simulink model "r2_b16a4x64f"  (R2012b)
settings: Solver=VariableStepDiscrete  SolverMode=SingleTasking  StartTime=0.0  StopTime=1  RelTol=1e-3
undefined symbols (not defined in the file): fft_stages, n_bits_ants, n_bits_xengs
libraries: xbsIndex_r4 x26846, casper_library_misc x230, xbsReplacements_r4 x24, casper_library_delays x8, xps_library x5, casper_library_communications x4
(part 25 of 227)

== system r2_b16a4x64f/vacc_monitor3 ==
  cnt_rst : Inport
  eof : Inport  Port=2
  error : Inport  Port=3
  Delay1 : Subsystem  AncestorBlock=casper_library_delays/pipeline  mask(pipeline){latency=2}
      mask help:
      | An explicitly laid-out delay line to avoid mapping to SRL16s
      | for use in pipelining to help achieve timing closure.
      mask init:
      | pipeline_init(gcb,'latency',latency);
      settings: AttributesFormatString=Latency = %<latency>
      mask Display:
      | port_label('input', 1, 'd');
      | port_label('output', 1, 'q');
      | disp(['Z^-', num2str(latency)]);
  Delay2 : Subsystem  AncestorBlock=casper_library_delays/pipeline  mask(pipeline){latency=2}
      mask help:
      | An explicitly laid-out delay line to avoid mapping to SRL16s
      | for use in pipelining to help achieve timing closure.
      mask init:
      | pipeline_init(gcb,'latency',latency);
      settings: AttributesFormatString=Latency = %<latency>
      mask Display:
      | port_label('input', 1, 'd');
      | port_label('output', 1, 'q');
      | disp(['Z^-', num2str(latency)]);
  Delay29 : Subsystem  AncestorBlock=casper_library_delays/pipeline  mask(pipeline){latency=2}
      mask help:
      | An explicitly laid-out delay line to avoid mapping to SRL16s
      | for use in pipelining to help achieve timing closure.
      mask init:
      | pipeline_init(gcb,'latency',latency);
      settings: AttributesFormatString=Latency = %<latency>
      mask Display:
      | port_label('input', 1, 'd');
      | port_label('output', 1, 'q');
      | disp(['Z^-', num2str(latency)]);
  Delay3 : Subsystem  AncestorBlock=casper_library_delays/pipeline  mask(pipeline){latency=2}
      mask help:
      | An explicitly laid-out delay line to avoid mapping to SRL16s
      | for use in pipelining to help achieve timing closure.
      mask init:
      | pipeline_init(gcb,'latency',latency);
      settings: AttributesFormatString=Latency = %<latency>
      mask Display:
      | port_label('input', 1, 'd');
      | port_label('output', 1, 'q');
      | disp(['Z^-', num2str(latency)]);
  Delay4 : Subsystem  AncestorBlock=casper_library_delays/pipeline  mask(pipeline){latency=2}
      mask help:
      | An explicitly laid-out delay line to avoid mapping to SRL16s
      | for use in pipelining to help achieve timing closure.
      mask init:
      | pipeline_init(gcb,'latency',latency);
      settings: AttributesFormatString=Latency = %<latency>
      mask Display:
      | port_label('input', 1, 'd');
      | port_label('output', 1, 'q');
      | disp(['Z^-', num2str(latency)]);
  payload_cnt1 : xbsIndex_r4/Counter  cnt_type=Free Running  cnt_to=0  operation=Up  start_count=0  cnt_by_val=1  arith_type=Unsigned  n_bits=16  bin_pt=0  load_pin=off  rst=on  en=on  explicit_period=off  period=1  dbl_ovrd=off  use_behavioral_HDL=on  implementation=Fabric  use_rpm=on  block_type=counter
      settings: xl_area=[0, 0, 0, 0, 0, 0, 0]
  payload_cnt3 : xbsIndex_r4/Counter  cnt_type=Free Running  cnt_to=0  operation=Up  start_count=0  cnt_by_val=1  arith_type=Unsigned  n_bits=16  bin_pt=0  load_pin=off  rst=on  en=on  explicit_period=off  period=1  dbl_ovrd=off  use_behavioral_HDL=on  implementation=Fabric  use_rpm=on  block_type=counter
      settings: xl_area=[0, 0, 0, 0, 0, 0, 0]
  pkt_cnt : Outport
  error_cnt : Outport  Port=2
  wires:
  Delay3/1(q) -> pkt_cnt/1
  error/1 -> Delay29/1(d)
  Delay4/1(q) -> error_cnt/1
  eof/1 -> Delay1/1(d)
  cnt_rst/1 -> Delay2/1(d)
  payload_cnt1/1 -> Delay4/1(d)
  Delay29/1(q) -> payload_cnt1/2
  Delay1/1(q) -> payload_cnt3/2
  Delay2/1(q) -> payload_cnt1/1, payload_cnt3/1
  payload_cnt3/1 -> Delay3/1(d)

== system r2_b16a4x64f/vacc_monitor4 ==
  cnt_rst : Inport
  new_acc : Inport  Port=2
  ready : Inport  Port=3
  eof : Inport  Port=4
  error : Inport  Port=5
  Delay1 : Subsystem  AncestorBlock=casper_library_delays/pipeline  mask(pipeline){latency=2}
      mask help:
      | An explicitly laid-out delay line to avoid mapping to SRL16s
      | for use in pipelining to help achieve timing closure.
      mask init:
      | pipeline_init(gcb,'latency',latency);
      settings: AttributesFormatString=Latency = %<latency>
      mask Display:
      | port_label('input', 1, 'd');
      | port_label('output', 1, 'q');
      | disp(['Z^-', num2str(latency)]);
  Delay121 : Subsystem  AncestorBlock=casper_library_delays/pipeline  mask(pipeline){latency=2}
      mask help:
      | An explicitly laid-out delay line to avoid mapping to SRL16s
      | for use in pipelining to help achieve timing closure.
      mask init:
      | pipeline_init(gcb,'latency',latency);
      settings: AttributesFormatString=Latency = %<latency>
      mask Display:
      | port_label('input', 1, 'd');
      | port_label('output', 1, 'q');
      | disp(['Z^-', num2str(latency)]);
  Delay2 : Subsystem  AncestorBlock=casper_library_delays/pipeline  mask(pipeline){latency=2}
      mask help:
      | An explicitly laid-out delay line to avoid mapping to SRL16s
      | for use in pipelining to help achieve timing closure.
      mask init:
      | pipeline_init(gcb,'latency',latency);
      settings: AttributesFormatString=Latency = %<latency>
      mask Display:
      | port_label('input', 1, 'd');
      | port_label('output', 1, 'q');
      | disp(['Z^-', num2str(latency)]);
  Delay25 : Subsystem  AncestorBlock=casper_library_delays/pipeline  mask(pipeline){latency=2}
      mask help:
      | An explicitly laid-out delay line to avoid mapping to SRL16s
      | for use in pipelining to help achieve timing closure.
      mask init:
      | pipeline_init(gcb,'latency',latency);
      settings: AttributesFormatString=Latency = %<latency>
      mask Display:
      | port_label('input', 1, 'd');
      | port_label('output', 1, 'q');
      | disp(['Z^-', num2str(latency)]);
  Delay3 : Subsystem  AncestorBlock=casper_library_delays/pipeline  mask(pipeline){latency=2}
      mask help:
      | An explicitly laid-out delay line to avoid mapping to SRL16s
      | for use in pipelining to help achieve timing closure.
      mask init:
      | pipeline_init(gcb,'latency',latency);
      settings: AttributesFormatString=Latency = %<latency>
      mask Display:
      | port_label('input', 1, 'd');
      | port_label('output', 1, 'q');
      | disp(['Z^-', num2str(latency)]);
  Delay4 : Subsystem  AncestorBlock=casper_library_delays/pipeline  mask(pipeline){latency=2}
      mask help:
      | An explicitly laid-out delay line to avoid mapping to SRL16s
      | for use in pipelining to help achieve timing closure.
      mask init:
      | pipeline_init(gcb,'latency',latency);
      settings: AttributesFormatString=Latency = %<latency>
      mask Display:
      | port_label('input', 1, 'd');
      | port_label('output', 1, 'q');
      | disp(['Z^-', num2str(latency)]);
  Delay5 : Subsystem  AncestorBlock=casper_library_delays/pipeline  mask(pipeline){latency=2}
      mask help:
      | An explicitly laid-out delay line to avoid mapping to SRL16s
      | for use in pipelining to help achieve timing closure.
      mask init:
      | pipeline_init(gcb,'latency',latency);
      settings: AttributesFormatString=Latency = %<latency>
      mask Display:
      | port_label('input', 1, 'd');
      | port_label('output', 1, 'q');
      | disp(['Z^-', num2str(latency)]);
  Delay6 : Subsystem  AncestorBlock=casper_library_delays/pipeline  mask(pipeline){latency=2}
      mask help:
      | An explicitly laid-out delay line to avoid mapping to SRL16s
      | for use in pipelining to help achieve timing closure.
      mask init:
      | pipeline_init(gcb,'latency',latency);
      settings: AttributesFormatString=Latency = %<latency>
      mask Display:
      | port_label('input', 1, 'd');
      | port_label('output', 1, 'q');
      | disp(['Z^-', num2str(latency)]);
  Delay7 : Subsystem  AncestorBlock=casper_library_delays/pipeline  mask(pipeline){latency=2}
      mask help:
      | An explicitly laid-out delay line to avoid mapping to SRL16s
      | for use in pipelining to help achieve timing closure.
      mask init:
      | pipeline_init(gcb,'latency',latency);
      settings: AttributesFormatString=Latency = %<latency>
      mask Display:
      | port_label('input', 1, 'd');
      | port_label('output', 1, 'q');
      | disp(['Z^-', num2str(latency)]);
  payload_cnt{1..4} (4 alike) : xbsIndex_r4/Counter  cnt_type=Free Running  cnt_to=0  operation=Up  start_count=0  cnt_by_val=1  arith_type=Unsigned  n_bits=16  bin_pt=0  load_pin=off  rst=on  en=on  explicit_period=off  period=1  dbl_ovrd=off  use_behavioral_HDL=on  implementation=Fabric  use_rpm=on  block_type=counter
      settings: xl_area=[0, 0, 0, 0, 0, 0, 0]
  acc_cnt : Outport
  ready_cnt : Outport  Port=2
  eof_cnt : Outport  Port=3
  error_cnt : Outport  Port=4
  wires:
  Delay5/1(q) -> eof_cnt/1
  Delay4/1(q) -> ready_cnt/1
  Delay7/1(q) -> payload_cnt2/2
  Delay6/1(q) -> payload_cnt4/2
  payload_cnt4/1 -> Delay5/1(d)
  payload_cnt2/1 -> Delay4/1(d)
  ready/1 -> Delay7/1(d)
  eof/1 -> Delay6/1(d)
  Delay3/1(q) -> payload_cnt3/1, payload_cnt2/1, payload_cnt4/1, payload_cnt1/1
  Delay121/1(q) -> acc_cnt/1
  error/1 -> Delay1/1(d)
  Delay25/1(q) -> error_cnt/1
  new_acc/1 -> Delay2/1(d)
  cnt_rst/1 -> Delay3/1(d)
  payload_cnt1/1 -> Delay25/1(d)
  Delay1/1(q) -> payload_cnt1/2
  payload_cnt3/1 -> Delay121/1(d)
  Delay2/1(q) -> payload_cnt3/2

== system r2_b16a4x64f/vacc_monitor5 ==
  cnt_rst : Inport
  eof : Inport  Port=2
  error : Inport  Port=3
  Delay1 : Subsystem  AncestorBlock=casper_library_delays/pipeline  mask(pipeline){latency=2}
      mask help:
      | An explicitly laid-out delay line to avoid mapping to SRL16s
      | for use in pipelining to help achieve timing closure.
      mask init:
      | pipeline_init(gcb,'latency',latency);
      settings: AttributesFormatString=Latency = %<latency>
      mask Display:
      | port_label('input', 1, 'd');
      | port_label('output', 1, 'q');
      | disp(['Z^-', num2str(latency)]);
  Delay2 : Subsystem  AncestorBlock=casper_library_delays/pipeline  mask(pipeline){latency=2}
      mask help:
      | An explicitly laid-out delay line to avoid mapping to SRL16s
      | for use in pipelining to help achieve timing closure.
      mask init:
      | pipeline_init(gcb,'latency',latency);
      settings: AttributesFormatString=Latency = %<latency>
      mask Display:
      | port_label('input', 1, 'd');
      | port_label('output', 1, 'q');
      | disp(['Z^-', num2str(latency)]);
  Delay29 : Subsystem  AncestorBlock=casper_library_delays/pipeline  mask(pipeline){latency=2}
      mask help:
      | An explicitly laid-out delay line to avoid mapping to SRL16s
      | for use in pipelining to help achieve timing closure.
      mask init:
      | pipeline_init(gcb,'latency',latency);
      settings: AttributesFormatString=Latency = %<latency>
      mask Display:
      | port_label('input', 1, 'd');
      | port_label('output', 1, 'q');
      | disp(['Z^-', num2str(latency)]);
  Delay3 : Subsystem  AncestorBlock=casper_library_delays/pipeline  mask(pipeline){latency=2}
      mask help:
      | An explicitly laid-out delay line to avoid mapping to SRL16s
      | for use in pipelining to help achieve timing closure.
      mask init:
      | pipeline_init(gcb,'latency',latency);
      settings: AttributesFormatString=Latency = %<latency>
      mask Display:
      | port_label('input', 1, 'd');
      | port_label('output', 1, 'q');
      | disp(['Z^-', num2str(latency)]);
  Delay4 : Subsystem  AncestorBlock=casper_library_delays/pipeline  mask(pipeline){latency=2}
      mask help:
      | An explicitly laid-out delay line to avoid mapping to SRL16s
      | for use in pipelining to help achieve timing closure.
      mask init:
      | pipeline_init(gcb,'latency',latency);
      settings: AttributesFormatString=Latency = %<latency>
      mask Display:
      | port_label('input', 1, 'd');
      | port_label('output', 1, 'q');
      | disp(['Z^-', num2str(latency)]);
  payload_cnt1 : xbsIndex_r4/Counter  cnt_type=Free Running  cnt_to=0  operation=Up  start_count=0  cnt_by_val=1  arith_type=Unsigned  n_bits=16  bin_pt=0  load_pin=off  rst=on  en=on  explicit_period=off  period=1  dbl_ovrd=off  use_behavioral_HDL=on  implementation=Fabric  use_rpm=on  block_type=counter
      settings: xl_area=[0, 0, 0, 0, 0, 0, 0]
  payload_cnt3 : xbsIndex_r4/Counter  cnt_type=Free Running  cnt_to=0  operation=Up  start_count=0  cnt_by_val=1  arith_type=Unsigned  n_bits=16  bin_pt=0  load_pin=off  rst=on  en=on  explicit_period=off  period=1  dbl_ovrd=off  use_behavioral_HDL=on  implementation=Fabric  use_rpm=on  block_type=counter
      settings: xl_area=[0, 0, 0, 0, 0, 0, 0]
  pkt_cnt : Outport
  error_cnt : Outport  Port=2
  wires:
  Delay3/1(q) -> pkt_cnt/1
  error/1 -> Delay29/1(d)
  Delay4/1(q) -> error_cnt/1
  eof/1 -> Delay1/1(d)
  cnt_rst/1 -> Delay2/1(d)
  payload_cnt1/1 -> Delay4/1(d)
  Delay29/1(q) -> payload_cnt1/2
  Delay1/1(q) -> payload_cnt3/2
  Delay2/1(q) -> payload_cnt1/1, payload_cnt3/1
  payload_cnt3/1 -> Delay3/1(d)

== system r2_b16a4x64f/vacc_monitor6 ==
  cnt_rst : Inport
  cal : Inport  Port=2
  inof : Inport  Port=3
  rst : Inport  Port=4
  outof : Inport  Port=5
  parity : Inport  Port=6
  Delay1 : Subsystem  AncestorBlock=casper_library_delays/pipeline  mask(pipeline){latency=2}
      mask help:
      | An explicitly laid-out delay line to avoid mapping to SRL16s
      | for use in pipelining to help achieve timing closure.
      mask init:
      | pipeline_init(gcb,'latency',latency);
      settings: AttributesFormatString=Latency = %<latency>
      mask Display:
      | port_label('input', 1, 'd');
      | port_label('output', 1, 'q');
      | disp(['Z^-', num2str(latency)]);
  Delay2 : Subsystem  AncestorBlock=casper_library_delays/pipeline  mask(pipeline){latency=2}
      mask help:
      | An explicitly laid-out delay line to avoid mapping to SRL16s
      | for use in pipelining to help achieve timing closure.
      mask init:
      | pipeline_init(gcb,'latency',latency);
      settings: AttributesFormatString=Latency = %<latency>
      mask Display:
      | port_label('input', 1, 'd');
      | port_label('output', 1, 'q');
      | disp(['Z^-', num2str(latency)]);
  Delay25 : Subsystem  AncestorBlock=casper_library_delays/pipeline  mask(pipeline){latency=2}
      mask help:
      | An explicitly laid-out delay line to avoid mapping to SRL16s
      | for use in pipelining to help achieve timing closure.
      mask init:
      | pipeline_init(gcb,'latency',latency);
      settings: AttributesFormatString=Latency = %<latency>
      mask Display:
      | port_label('input', 1, 'd');
      | port_label('output', 1, 'q');
      | disp(['Z^-', num2str(latency)]);
  Delay3 : Subsystem  AncestorBlock=casper_library_delays/pipeline  mask(pipeline){latency=2}
      mask help:
      | An explicitly laid-out delay line to avoid mapping to SRL16s
      | for use in pipelining to help achieve timing closure.
      mask init:
      | pipeline_init(gcb,'latency',latency);
      settings: AttributesFormatString=Latency = %<latency>
      mask Display:
      | port_label('input', 1, 'd');
      | port_label('output', 1, 'q');
      | disp(['Z^-', num2str(latency)]);
  Delay4 : Subsystem  AncestorBlock=casper_library_delays/pipeline  mask(pipeline){latency=2}
      mask help:
      | An explicitly laid-out delay line to avoid mapping to SRL16s
      | for use in pipelining to help achieve timing closure.
      mask init:
      | pipeline_init(gcb,'latency',latency);
      settings: AttributesFormatString=Latency = %<latency>
      mask Display:
      | port_label('input', 1, 'd');
      | port_label('output', 1, 'q');
      | disp(['Z^-', num2str(latency)]);
  payload_cnt{1..5} (5 alike) : xbsIndex_r4/Counter  cnt_type=Free Running  cnt_to=0  operation=Up  start_count=0  cnt_by_val=1  arith_type=Unsigned  n_bits=6  bin_pt=0  load_pin=off  rst=on  en=on  explicit_period=off  period=1  dbl_ovrd=off  use_behavioral_HDL=off  implementation=Fabric  use_rpm=on  block_type=counter
      settings: xl_area=[0, 0, 0, 0, 0, 0, 0]
  cal_cnt : Outport
  inof_cnt : Outport  Port=2
  rst_cnt : Outport  Port=3
  outof_cnt : Outport  Port=4
  parity_cnt : Outport  Port=5
  wires:
  Delay25/1(q) -> cal_cnt/1
  inof/1 -> payload_cnt3/2
  cnt_rst/1 -> payload_cnt1/1, payload_cnt2/1, payload_cnt4/1, payload_cnt5/1, payload_cnt3/1
  payload_cnt1/1 -> Delay25/1(d)
  cal/1 -> payload_cnt1/2
  payload_cnt3/1 -> Delay1/1(d)
  rst/1 -> payload_cnt2/2
  outof/1 -> payload_cnt4/2
  payload_cnt2/1 -> Delay2/1(d)
  payload_cnt4/1 -> Delay3/1(d)
  parity/1 -> payload_cnt5/2
  payload_cnt5/1 -> Delay4/1(d)
  Delay1/1(q) -> inof_cnt/1
  Delay2/1(q) -> rst_cnt/1
  Delay3/1(q) -> outof_cnt/1
  Delay4/1(q) -> parity_cnt/1

== system r2_b16a4x64f/vacc_monitor7 ==
  cnt_rst : Inport
  eof : Inport  Port=2
  error : Inport  Port=3
  Delay1 : Subsystem  AncestorBlock=casper_library_delays/pipeline  mask(pipeline){latency=2}
      mask help:
      | An explicitly laid-out delay line to avoid mapping to SRL16s
      | for use in pipelining to help achieve timing closure.
      mask init:
      | pipeline_init(gcb,'latency',latency);
      settings: AttributesFormatString=Latency = %<latency>
      mask Display:
      | port_label('input', 1, 'd');
      | port_label('output', 1, 'q');
      | disp(['Z^-', num2str(latency)]);
  Delay2 : Subsystem  AncestorBlock=casper_library_delays/pipeline  mask(pipeline){latency=2}
      mask help:
      | An explicitly laid-out delay line to avoid mapping to SRL16s
      | for use in pipelining to help achieve timing closure.
      mask init:
      | pipeline_init(gcb,'latency',latency);
      settings: AttributesFormatString=Latency = %<latency>
      mask Display:
      | port_label('input', 1, 'd');
      | port_label('output', 1, 'q');
      | disp(['Z^-', num2str(latency)]);
  Delay29 : Subsystem  AncestorBlock=casper_library_delays/pipeline  mask(pipeline){latency=2}
      mask help:
      | An explicitly laid-out delay line to avoid mapping to SRL16s
      | for use in pipelining to help achieve timing closure.
      mask init:
      | pipeline_init(gcb,'latency',latency);
      settings: AttributesFormatString=Latency = %<latency>
      mask Display:
      | port_label('input', 1, 'd');
      | port_label('output', 1, 'q');
      | disp(['Z^-', num2str(latency)]);
  Delay3 : Subsystem  AncestorBlock=casper_library_delays/pipeline  mask(pipeline){latency=2}
      mask help:
      | An explicitly laid-out delay line to avoid mapping to SRL16s
      | for use in pipelining to help achieve timing closure.
      mask init:
      | pipeline_init(gcb,'latency',latency);
      settings: AttributesFormatString=Latency = %<latency>
      mask Display:
      | port_label('input', 1, 'd');
      | port_label('output', 1, 'q');
      | disp(['Z^-', num2str(latency)]);
  Delay4 : Subsystem  AncestorBlock=casper_library_delays/pipeline  mask(pipeline){latency=2}
      mask help:
      | An explicitly laid-out delay line to avoid mapping to SRL16s
      | for use in pipelining to help achieve timing closure.
      mask init:
      | pipeline_init(gcb,'latency',latency);
      settings: AttributesFormatString=Latency = %<latency>
      mask Display:
      | port_label('input', 1, 'd');
      | port_label('output', 1, 'q');
      | disp(['Z^-', num2str(latency)]);
  payload_cnt1 : xbsIndex_r4/Counter  cnt_type=Free Running  cnt_to=0  operation=Up  start_count=0  cnt_by_val=1  arith_type=Unsigned  n_bits=16  bin_pt=0  load_pin=off  rst=on  en=on  explicit_period=off  period=1  dbl_ovrd=off  use_behavioral_HDL=on  implementation=Fabric  use_rpm=on  block_type=counter
      settings: xl_area=[0, 0, 0, 0, 0, 0, 0]
  payload_cnt3 : xbsIndex_r4/Counter  cnt_type=Free Running  cnt_to=0  operation=Up  start_count=0  cnt_by_val=1  arith_type=Unsigned  n_bits=16  bin_pt=0  load_pin=off  rst=on  en=on  explicit_period=off  period=1  dbl_ovrd=off  use_behavioral_HDL=on  implementation=Fabric  use_rpm=on  block_type=counter
      settings: xl_area=[0, 0, 0, 0, 0, 0, 0]
  pkt_cnt : Outport
  error_cnt : Outport  Port=2
  wires:
  payload_cnt3/1 -> Delay3/1(d)
  Delay2/1(q) -> payload_cnt3/1, payload_cnt1/1
  Delay1/1(q) -> payload_cnt3/2
  Delay29/1(q) -> payload_cnt1/2
  payload_cnt1/1 -> Delay4/1(d)
  cnt_rst/1 -> Delay2/1(d)
  eof/1 -> Delay1/1(d)
  Delay4/1(q) -> error_cnt/1
  error/1 -> Delay29/1(d)
  Delay3/1(q) -> pkt_cnt/1

== system r2_b16a4x64f/vacc_monitor8 ==
  cnt_rst : Inport
  cal : Inport  Port=2
  inof : Inport  Port=3
  rst : Inport  Port=4
  outof : Inport  Port=5
  parity : Inport  Port=6
  Delay1 : Subsystem  AncestorBlock=casper_library_delays/pipeline  mask(pipeline){latency=2}
      mask help:
      | An explicitly laid-out delay line to avoid mapping to SRL16s
      | for use in pipelining to help achieve timing closure.
      mask init:
      | pipeline_init(gcb,'latency',latency);
      settings: AttributesFormatString=Latency = %<latency>
      mask Display:
      | port_label('input', 1, 'd');
      | port_label('output', 1, 'q');
      | disp(['Z^-', num2str(latency)]);
  Delay10 : Subsystem  AncestorBlock=casper_library_delays/pipeline  mask(pipeline){latency=2}
      mask help:
      | An explicitly laid-out delay line to avoid mapping to SRL16s
      | for use in pipelining to help achieve timing closure.
      mask init:
      | pipeline_init(gcb,'latency',latency);
      settings: AttributesFormatString=Latency = %<latency>
      mask Display:
      | port_label('input', 1, 'd');
      | port_label('output', 1, 'q');
      | disp(['Z^-', num2str(latency)]);
  Delay2 : Subsystem  AncestorBlock=casper_library_delays/pipeline  mask(pipeline){latency=2}
      mask help:
      | An explicitly laid-out delay line to avoid mapping to SRL16s
      | for use in pipelining to help achieve timing closure.
      mask init:
      | pipeline_init(gcb,'latency',latency);
      settings: AttributesFormatString=Latency = %<latency>
      mask Display:
      | port_label('input', 1, 'd');
      | port_label('output', 1, 'q');
      | disp(['Z^-', num2str(latency)]);
  Delay29 : Subsystem  AncestorBlock=casper_library_delays/pipeline  mask(pipeline){latency=2}
      mask help:
      | An explicitly laid-out delay line to avoid mapping to SRL16s
      | for use in pipelining to help achieve timing closure.
      mask init:
      | pipeline_init(gcb,'latency',latency);
      settings: AttributesFormatString=Latency = %<latency>
      mask Display:
      | port_label('input', 1, 'd');
      | port_label('output', 1, 'q');
      | disp(['Z^-', num2str(latency)]);
  Delay3 : Subsystem  AncestorBlock=casper_library_delays/pipeline  mask(pipeline){latency=2}
      mask help:
      | An explicitly laid-out delay line to avoid mapping to SRL16s
      | for use in pipelining to help achieve timing closure.
      mask init:
      | pipeline_init(gcb,'latency',latency);
      settings: AttributesFormatString=Latency = %<latency>
      mask Display:
      | port_label('input', 1, 'd');
      | port_label('output', 1, 'q');
      | disp(['Z^-', num2str(latency)]);
  Delay4 : Subsystem  AncestorBlock=casper_library_delays/pipeline  mask(pipeline){latency=2}
      mask help:
      | An explicitly laid-out delay line to avoid mapping to SRL16s
      | for use in pipelining to help achieve timing closure.
      mask init:
      | pipeline_init(gcb,'latency',latency);
      settings: AttributesFormatString=Latency = %<latency>
      mask Display:
      | port_label('input', 1, 'd');
      | port_label('output', 1, 'q');
      | disp(['Z^-', num2str(latency)]);
  Delay5 : Subsystem  AncestorBlock=casper_library_delays/pipeline  mask(pipeline){latency=2}
      mask help:
      | An explicitly laid-out delay line to avoid mapping to SRL16s
      | for use in pipelining to help achieve timing closure.
      mask init:
      | pipeline_init(gcb,'latency',latency);
      settings: AttributesFormatString=Latency = %<latency>
      mask Display:
      | port_label('input', 1, 'd');
      | port_label('output', 1, 'q');
      | disp(['Z^-', num2str(latency)]);
  Delay6 : Subsystem  AncestorBlock=casper_library_delays/pipeline  mask(pipeline){latency=2}
      mask help:
      | An explicitly laid-out delay line to avoid mapping to SRL16s
      | for use in pipelining to help achieve timing closure.
      mask init:
      | pipeline_init(gcb,'latency',latency);
      settings: AttributesFormatString=Latency = %<latency>
      mask Display:
      | port_label('input', 1, 'd');
      | port_label('output', 1, 'q');
      | disp(['Z^-', num2str(latency)]);
  Delay7 : Subsystem  AncestorBlock=casper_library_delays/pipeline  mask(pipeline){latency=2}
      mask help:
      | An explicitly laid-out delay line to avoid mapping to SRL16s
      | for use in pipelining to help achieve timing closure.
      mask init:
      | pipeline_init(gcb,'latency',latency);
      settings: AttributesFormatString=Latency = %<latency>
      mask Display:
      | port_label('input', 1, 'd');
      | port_label('output', 1, 'q');
      | disp(['Z^-', num2str(latency)]);
  Delay8 : Subsystem  AncestorBlock=casper_library_delays/pipeline  mask(pipeline){latency=2}
      mask help:
      | An explicitly laid-out delay line to avoid mapping to SRL16s
      | for use in pipelining to help achieve timing closure.
      mask init:
      | pipeline_init(gcb,'latency',latency);
      settings: AttributesFormatString=Latency = %<latency>
      mask Display:
      | port_label('input', 1, 'd');
      | port_label('output', 1, 'q');
      | disp(['Z^-', num2str(latency)]);
  Delay9 : Subsystem  AncestorBlock=casper_library_delays/pipeline  mask(pipeline){latency=2}
      mask help:
      | An explicitly laid-out delay line to avoid mapping to SRL16s
      | for use in pipelining to help achieve timing closure.
      mask init:
      | pipeline_init(gcb,'latency',latency);
      settings: AttributesFormatString=Latency = %<latency>
      mask Display:
      | port_label('input', 1, 'd');
      | port_label('output', 1, 'q');
      | disp(['Z^-', num2str(latency)]);
  payload_cnt{1..5} (5 alike) : xbsIndex_r4/Counter  cnt_type=Free Running  cnt_to=0  operation=Up  start_count=0  cnt_by_val=1  arith_type=Unsigned  n_bits=6  bin_pt=0  load_pin=off  rst=on  en=on  explicit_period=off  period=1  dbl_ovrd=off  use_behavioral_HDL=off  implementation=Fabric  use_rpm=on  block_type=counter
      settings: xl_area=[0, 0, 0, 0, 0, 0, 0]
  cal_cnt : Outport
  inof_cnt : Outport  Port=2
  rst_cnt : Outport  Port=3
  outof_cnt : Outport  Port=4
  parity_cnt : Outport  Port=5
  wires:
  cal/1 -> Delay29/1(d)
  inof/1 -> Delay8/1(d)
  cnt_rst/1 -> Delay2/1(d)
  payload_cnt1/1 -> Delay1/1(d)
  Delay29/1(q) -> payload_cnt1/2
  rst/1 -> Delay7/1(d)
  outof/1 -> Delay9/1(d)
  parity/1 -> Delay10/1(d)
  Delay2/1(q) -> payload_cnt1/1, payload_cnt2/1, payload_cnt4/1, payload_cnt5/1, payload_cnt3/1
  payload_cnt3/1 -> Delay3/1(d)
  payload_cnt2/1 -> Delay4/1(d)
  payload_cnt4/1 -> Delay5/1(d)
  payload_cnt5/1 -> Delay6/1(d)
  Delay3/1(q) -> inof_cnt/1
  Delay1/1(q) -> cal_cnt/1
  Delay4/1(q) -> rst_cnt/1
  Delay5/1(q) -> outof_cnt/1
  Delay6/1(q) -> parity_cnt/1
  Delay10/1(q) -> payload_cnt5/2
  Delay9/1(q) -> payload_cnt4/2
  Delay7/1(q) -> payload_cnt2/2
  Delay8/1(q) -> payload_cnt3/2

== system r2_b16a4x64f/vacc_monitor9 ==
  cnt_rst : Inport
  cal : Inport  Port=2
  inof : Inport  Port=3
  rst : Inport  Port=4
  outof : Inport  Port=5
  parity : Inport  Port=6
  Delay1 : Subsystem  AncestorBlock=casper_library_delays/pipeline  mask(pipeline){latency=2}
      mask help:
      | An explicitly laid-out delay line to avoid mapping to SRL16s
      | for use in pipelining to help achieve timing closure.
      mask init:
      | pipeline_init(gcb,'latency',latency);
      settings: AttributesFormatString=Latency = %<latency>
      mask Display:
      | port_label('input', 1, 'd');
      | port_label('output', 1, 'q');
      | disp(['Z^-', num2str(latency)]);
  Delay10 : Subsystem  AncestorBlock=casper_library_delays/pipeline  mask(pipeline){latency=2}
      mask help:
      | An explicitly laid-out delay line to avoid mapping to SRL16s
      | for use in pipelining to help achieve timing closure.
      mask init:
      | pipeline_init(gcb,'latency',latency);
      settings: AttributesFormatString=Latency = %<latency>
      mask Display:
      | port_label('input', 1, 'd');
      | port_label('output', 1, 'q');
      | disp(['Z^-', num2str(latency)]);
  Delay2 : Subsystem  AncestorBlock=casper_library_delays/pipeline  mask(pipeline){latency=2}
      mask help:
      | An explicitly laid-out delay line to avoid mapping to SRL16s
      | for use in pipelining to help achieve timing closure.
      mask init:
      | pipeline_init(gcb,'latency',latency);
      settings: AttributesFormatString=Latency = %<latency>
      mask Display:
      | port_label('input', 1, 'd');
      | port_label('output', 1, 'q');
      | disp(['Z^-', num2str(latency)]);
  Delay29 : Subsystem  AncestorBlock=casper_library_delays/pipeline  mask(pipeline){latency=2}
      mask help:
      | An explicitly laid-out delay line to avoid mapping to SRL16s
      | for use in pipelining to help achieve timing closure.
      mask init:
      | pipeline_init(gcb,'latency',latency);
      settings: AttributesFormatString=Latency = %<latency>
      mask Display:
      | port_label('input', 1, 'd');
      | port_label('output', 1, 'q');
      | disp(['Z^-', num2str(latency)]);
  Delay3 : Subsystem  AncestorBlock=casper_library_delays/pipeline  mask(pipeline){latency=2}
      mask help:
      | An explicitly laid-out delay line to avoid mapping to SRL16s
      | for use in pipelining to help achieve timing closure.
      mask init:
      | pipeline_init(gcb,'latency',latency);
      settings: AttributesFormatString=Latency = %<latency>
      mask Display:
      | port_label('input', 1, 'd');
      | port_label('output', 1, 'q');
      | disp(['Z^-', num2str(latency)]);
  Delay4 : Subsystem  AncestorBlock=casper_library_delays/pipeline  mask(pipeline){latency=2}
      mask help:
      | An explicitly laid-out delay line to avoid mapping to SRL16s
      | for use in pipelining to help achieve timing closure.
      mask init:
      | pipeline_init(gcb,'latency',latency);
      settings: AttributesFormatString=Latency = %<latency>
      mask Display:
      | port_label('input', 1, 'd');
      | port_label('output', 1, 'q');
      | disp(['Z^-', num2str(latency)]);
  Delay5 : Subsystem  AncestorBlock=casper_library_delays/pipeline  mask(pipeline){latency=2}
      mask help:
      | An explicitly laid-out delay line to avoid mapping to SRL16s
      | for use in pipelining to help achieve timing closure.
      mask init:
      | pipeline_init(gcb,'latency',latency);
      settings: AttributesFormatString=Latency = %<latency>
      mask Display:
      | port_label('input', 1, 'd');
      | port_label('output', 1, 'q');
      | disp(['Z^-', num2str(latency)]);
  Delay6 : Subsystem  AncestorBlock=casper_library_delays/pipeline  mask(pipeline){latency=2}
      mask help:
      | An explicitly laid-out delay line to avoid mapping to SRL16s
      | for use in pipelining to help achieve timing closure.
      mask init:
      | pipeline_init(gcb,'latency',latency);
      settings: AttributesFormatString=Latency = %<latency>
      mask Display:
      | port_label('input', 1, 'd');
      | port_label('output', 1, 'q');
      | disp(['Z^-', num2str(latency)]);
  Delay7 : Subsystem  AncestorBlock=casper_library_delays/pipeline  mask(pipeline){latency=2}
      mask help:
      | An explicitly laid-out delay line to avoid mapping to SRL16s
      | for use in pipelining to help achieve timing closure.
      mask init:
      | pipeline_init(gcb,'latency',latency);
      settings: AttributesFormatString=Latency = %<latency>
      mask Display:
      | port_label('input', 1, 'd');
      | port_label('output', 1, 'q');
      | disp(['Z^-', num2str(latency)]);
  Delay8 : Subsystem  AncestorBlock=casper_library_delays/pipeline  mask(pipeline){latency=2}
      mask help:
      | An explicitly laid-out delay line to avoid mapping to SRL16s
      | for use in pipelining to help achieve timing closure.
      mask init:
      | pipeline_init(gcb,'latency',latency);
      settings: AttributesFormatString=Latency = %<latency>
      mask Display:
      | port_label('input', 1, 'd');
      | port_label('output', 1, 'q');
      | disp(['Z^-', num2str(latency)]);
  Delay9 : Subsystem  AncestorBlock=casper_library_delays/pipeline  mask(pipeline){latency=2}
      mask help:
      | An explicitly laid-out delay line to avoid mapping to SRL16s
      | for use in pipelining to help achieve timing closure.
      mask init:
      | pipeline_init(gcb,'latency',latency);
      settings: AttributesFormatString=Latency = %<latency>
      mask Display:
      | port_label('input', 1, 'd');
      | port_label('output', 1, 'q');
      | disp(['Z^-', num2str(latency)]);
  payload_cnt{1..5} (5 alike) : xbsIndex_r4/Counter  cnt_type=Free Running  cnt_to=0  operation=Up  start_count=0  cnt_by_val=1  arith_type=Unsigned  n_bits=6  bin_pt=0  load_pin=off  rst=on  en=on  explicit_period=off  period=1  dbl_ovrd=off  use_behavioral_HDL=off  implementation=Fabric  use_rpm=on  block_type=counter
      settings: xl_area=[0, 0, 0, 0, 0, 0, 0]
  cal_cnt : Outport
  inof_cnt : Outport  Port=2
  rst_cnt : Outport  Port=3
  outof_cnt : Outport  Port=4
  parity_cnt : Outport  Port=5
  wires:
  Delay8/1(q) -> payload_cnt3/2
  Delay7/1(q) -> payload_cnt2/2
  Delay9/1(q) -> payload_cnt4/2
  Delay10/1(q) -> payload_cnt5/2
  Delay6/1(q) -> parity_cnt/1
  Delay5/1(q) -> outof_cnt/1
  Delay4/1(q) -> rst_cnt/1
  Delay1/1(q) -> cal_cnt/1
  Delay3/1(q) -> inof_cnt/1
  payload_cnt5/1 -> Delay6/1(d)
  payload_cnt4/1 -> Delay5/1(d)
  payload_cnt2/1 -> Delay4/1(d)
  payload_cnt3/1 -> Delay3/1(d)
  Delay2/1(q) -> payload_cnt3/1, payload_cnt5/1, payload_cnt4/1, payload_cnt2/1, payload_cnt1/1
  parity/1 -> Delay10/1(d)
  outof/1 -> Delay9/1(d)
  rst/1 -> Delay7/1(d)
  Delay29/1(q) -> payload_cnt1/2
  payload_cnt1/1 -> Delay1/1(d)
  cnt_rst/1 -> Delay2/1(d)
  inof/1 -> Delay8/1(d)
  cal/1 -> Delay29/1(d)

== system r2_b16a4x64f/vacc_time_lsw ==
  io_delay : xbsIndex_r4/Delay  rst=off  infoeditControl=Selection of Reset will increase slice count due to use of real FFs and instead of SRLs  en=off  latency=0  dbl_ovrd=off  reg_retiming=on  block_type=delay
  r2_b16a4x64f_vacc_time_lsw_user_data_out : xbsIndex_r4/Gateway In  gui_display_data_type=Fixed-point  arith_type=Unsigned  n_bits=32  bin_pt=0  preci_type=Single  exp_width=8  frac_width=24  quantization="Round  (unbiased: +/- Inf)"  overflow=Saturate  period=1  dbl_ovrd=off  timing_constraint=None  locs_specified=off  LOCs={}  UseAsADC=off  ADCChannel='1'  inherit_from_input=off  hdl_port=on  block_type=gatewayin
  reint1 : xbsIndex_r4/Reinterpret  force_arith_type=on  arith_type=Unsigned  force_bin_pt=on  bin_pt=0  block_type=reinterpret
  sim_1 : Constant  Value=0
  slice_lsw : xbsIndex_r4/Slice  nbits=32  boolean_output=off  mode=Lower Bit Location + Width  bit1=0  base1=MSB of Input  bit0=0  base0=LSB of Input  dbl_ovrd=off  block_type=slice
  in_lsw : Outport
  wires:
  r2_b16a4x64f_vacc_time_lsw_user_data_out/1 -> io_delay/1
  sim_1/1 -> r2_b16a4x64f_vacc_time_lsw_user_data_out/1
  io_delay/1 -> slice_lsw/1
  slice_lsw/1 -> reint1/1
  reint1/1 -> in_lsw/1

== system r2_b16a4x64f/vacc_time_msw ==
  convert1_1 : DataTypeConversion  OutDataTypeStr=fixdt('ufix1_En0')  LockScale=on
  convert1_2 : DataTypeConversion  OutDataTypeStr=fixdt('ufix1_En0')  LockScale=on
  convert1_3 : DataTypeConversion  OutDataTypeStr=fixdt('ufix16_En0')  LockScale=on
  convert2_1 : DataTypeConversion  OutDataTypeStr=fixdt('ufix1_En0')  ConvertRealWorld=Stored Integer (SI)  LockScale=on
  convert2_2 : DataTypeConversion  OutDataTypeStr=fixdt('ufix1_En0')  ConvertRealWorld=Stored Integer (SI)  LockScale=on
  convert2_3 : DataTypeConversion  OutDataTypeStr=fixdt('ufix16_En0')  ConvertRealWorld=Stored Integer (SI)  LockScale=on
  gain_1 : Gain  Gain=131072
  gain_2 : Gain  Gain=65536
  gain_3 : Gain
  io_delay : xbsIndex_r4/Delay  rst=off  infoeditControl=Selection of Reset will increase slice count due to use of real FFs and instead of SRLs  en=off  latency=0  dbl_ovrd=off  reg_retiming=on  block_type=delay
  r2_b16a4x64f_vacc_time_msw_user_data_out : xbsIndex_r4/Gateway In  gui_display_data_type=Fixed-point  arith_type=Unsigned  n_bits=32  bin_pt=0  preci_type=Single  exp_width=8  frac_width=24  quantization="Round  (unbiased: +/- Inf)"  overflow=Saturate  period=1  dbl_ovrd=off  timing_constraint=None  locs_specified=off  LOCs={}  UseAsADC=off  ADCChannel='1'  inherit_from_input=off  hdl_port=on  block_type=gatewayin
  reint3 : xbsIndex_r4/Reinterpret  force_arith_type=on  arith_type=Unsigned  force_bin_pt=on  bin_pt=0  block_type=reinterpret
  sim_1 : Constant  Value=0
  sim_2 : Constant  Value=0
  sim_3 : Constant  Value=0
  sim_add : Sum  Inputs=+++  OutDataTypeStr=uint32
  slice_arm : xbsIndex_r4/Slice  nbits=1  boolean_output=on  mode=Lower Bit Location + Width  bit1=0  base1=MSB of Input  bit0=17  base0=LSB of Input  dbl_ovrd=off  block_type=slice
  slice_immediate : xbsIndex_r4/Slice  nbits=1  boolean_output=on  mode=Lower Bit Location + Width  bit1=0  base1=MSB of Input  bit0=16  base0=LSB of Input  dbl_ovrd=off  block_type=slice
  slice_msw : xbsIndex_r4/Slice  nbits=16  boolean_output=off  mode=Lower Bit Location + Width  bit1=0  base1=MSB of Input  bit0=0  base0=LSB of Input  dbl_ovrd=off  block_type=slice
  in_arm : Outport
  in_immediate : Outport  Port=2
  in_msw : Outport  Port=3
  wires:
  r2_b16a4x64f_vacc_time_msw_user_data_out/1 -> io_delay/1
  sim_add/1 -> r2_b16a4x64f_vacc_time_msw_user_data_out/1
  sim_1/1 -> convert1_1/1
  convert1_1/1 -> convert2_1/1
  convert2_1/1 -> gain_1/1
  gain_1/1 -> sim_add/1
  io_delay/1 -> slice_arm/1, slice_immediate/1, slice_msw/1
  slice_arm/1 -> in_arm/1
  sim_2/1 -> convert1_2/1
  convert1_2/1 -> convert2_2/1
  convert2_2/1 -> gain_2/1
  gain_2/1 -> sim_add/2
  slice_immediate/1 -> in_immediate/1
  sim_3/1 -> convert1_3/1
  convert1_3/1 -> convert2_3/1
  convert2_3/1 -> gain_3/1
  gain_3/1 -> sim_add/3
  slice_msw/1 -> reint3/1
  reint3/1 -> in_msw/1

== system r2_b16a4x64f/vacccnt0 ==
  out_reg : Inport
  assert_reg : xbsIndex_r4/Assert  assert_type=on  type_source=Explicitly  gui_display_data_type=Fixed-point  arith_type=Unsigned  n_bits=16  bin_pt=0  preci_type=Single  exp_width=8  frac_width=24  assert_rate=off  rate_source=Explicitly  period=1  output_port=on  block_type=assert
  cast_gw : xbsIndex_r4/Convert  gui_display_data_type=Fixed-point  arith_type=Unsigned  n_bits=32  bin_pt=0  float_type=Single  exp_bits=8  fraction_bits=24  quantization=Truncate  overflow=Wrap  en=off  latency=0  dbl_ovrd=off  pipeline=off  block_type=convert
  io_delay : xbsIndex_r4/Delay  rst=off  infoeditControl=Selection of Reset will increase slice count due to use of real FFs and instead of SRLs  en=off  latency=1  dbl_ovrd=off  reg_retiming=on  block_type=delay
  r2_b16a4x64f_vacccnt0_user_data_in : xbsIndex_r4/Gateway Out  inherit_from_input=off  hdl_port=on  timing_constraint=None  locs_specified=off  LOCs={}  UseAsDAC=off  DACChannel='1'  block_type=gatewayout
  reint1 : xbsIndex_r4/Reinterpret  force_arith_type=on  arith_type=Unsigned  force_bin_pt=on  bin_pt=0  block_type=reinterpret
  sim_out : Terminator
  wires:
  io_delay/1 -> cast_gw/1
  cast_gw/1 -> r2_b16a4x64f_vacccnt0_user_data_in/1
  r2_b16a4x64f_vacccnt0_user_data_in/1 -> sim_out/1
  out_reg/1 -> assert_reg/1
  assert_reg/1 -> reint1/1
  reint1/1 -> io_delay/1

== system r2_b16a4x64f/vacccnt1 ==
  out_reg : Inport
  assert_reg : xbsIndex_r4/Assert  assert_type=on  type_source=Explicitly  gui_display_data_type=Fixed-point  arith_type=Unsigned  n_bits=16  bin_pt=0  preci_type=Single  exp_width=8  frac_width=24  assert_rate=off  rate_source=Explicitly  period=1  output_port=on  block_type=assert
  cast_gw : xbsIndex_r4/Convert  gui_display_data_type=Fixed-point  arith_type=Unsigned  n_bits=32  bin_pt=0  float_type=Single  exp_bits=8  fraction_bits=24  quantization=Truncate  overflow=Wrap  en=off  latency=0  dbl_ovrd=off  pipeline=off  block_type=convert
  io_delay : xbsIndex_r4/Delay  rst=off  infoeditControl=Selection of Reset will increase slice count due to use of real FFs and instead of SRLs  en=off  latency=1  dbl_ovrd=off  reg_retiming=on  block_type=delay
  r2_b16a4x64f_vacccnt1_user_data_in : xbsIndex_r4/Gateway Out  inherit_from_input=off  hdl_port=on  timing_constraint=None  locs_specified=off  LOCs={}  UseAsDAC=off  DACChannel='1'  block_type=gatewayout
  reint1 : xbsIndex_r4/Reinterpret  force_arith_type=on  arith_type=Unsigned  force_bin_pt=on  bin_pt=0  block_type=reinterpret
  sim_out : Terminator
  wires:
  io_delay/1 -> cast_gw/1
  cast_gw/1 -> r2_b16a4x64f_vacccnt1_user_data_in/1
  r2_b16a4x64f_vacccnt1_user_data_in/1 -> sim_out/1
  out_reg/1 -> assert_reg/1
  assert_reg/1 -> reint1/1
  reint1/1 -> io_delay/1

== system r2_b16a4x64f/vacccnt2 ==
  out_reg : Inport
  assert_reg : xbsIndex_r4/Assert  assert_type=on  type_source=Explicitly  gui_display_data_type=Fixed-point  arith_type=Unsigned  n_bits=16  bin_pt=0  preci_type=Single  exp_width=8  frac_width=24  assert_rate=off  rate_source=Explicitly  period=1  output_port=on  block_type=assert
  cast_gw : xbsIndex_r4/Convert  gui_display_data_type=Fixed-point  arith_type=Unsigned  n_bits=32  bin_pt=0  float_type=Single  exp_bits=8  fraction_bits=24  quantization=Truncate  overflow=Wrap  en=off  latency=0  dbl_ovrd=off  pipeline=off  block_type=convert
  io_delay : xbsIndex_r4/Delay  rst=off  infoeditControl=Selection of Reset will increase slice count due to use of real FFs and instead of SRLs  en=off  latency=1  dbl_ovrd=off  reg_retiming=on  block_type=delay
  r2_b16a4x64f_vacccnt2_user_data_in : xbsIndex_r4/Gateway Out  inherit_from_input=off  hdl_port=on  timing_constraint=None  locs_specified=off  LOCs={}  UseAsDAC=off  DACChannel='1'  block_type=gatewayout
  reint1 : xbsIndex_r4/Reinterpret  force_arith_type=on  arith_type=Unsigned  force_bin_pt=on  bin_pt=0  block_type=reinterpret
  sim_out : Terminator
  wires:
  io_delay/1 -> cast_gw/1
  cast_gw/1 -> r2_b16a4x64f_vacccnt2_user_data_in/1
  r2_b16a4x64f_vacccnt2_user_data_in/1 -> sim_out/1
  out_reg/1 -> assert_reg/1
  assert_reg/1 -> reint1/1
  reint1/1 -> io_delay/1

== system r2_b16a4x64f/vacccnt3 ==
  out_reg : Inport
  assert_reg : xbsIndex_r4/Assert  assert_type=on  type_source=Explicitly  gui_display_data_type=Fixed-point  arith_type=Unsigned  n_bits=16  bin_pt=0  preci_type=Single  exp_width=8  frac_width=24  assert_rate=off  rate_source=Explicitly  period=1  output_port=on  block_type=assert
  cast_gw : xbsIndex_r4/Convert  gui_display_data_type=Fixed-point  arith_type=Unsigned  n_bits=32  bin_pt=0  float_type=Single  exp_bits=8  fraction_bits=24  quantization=Truncate  overflow=Wrap  en=off  latency=0  dbl_ovrd=off  pipeline=off  block_type=convert
  io_delay : xbsIndex_r4/Delay  rst=off  infoeditControl=Selection of Reset will increase slice count due to use of real FFs and instead of SRLs  en=off  latency=1  dbl_ovrd=off  reg_retiming=on  block_type=delay
  r2_b16a4x64f_vacccnt3_user_data_in : xbsIndex_r4/Gateway Out  inherit_from_input=off  hdl_port=on  timing_constraint=None  locs_specified=off  LOCs={}  UseAsDAC=off  DACChannel='1'  block_type=gatewayout
  reint1 : xbsIndex_r4/Reinterpret  force_arith_type=on  arith_type=Unsigned  force_bin_pt=on  bin_pt=0  block_type=reinterpret
  sim_out : Terminator
  wires:
  io_delay/1 -> cast_gw/1
  cast_gw/1 -> r2_b16a4x64f_vacccnt3_user_data_in/1
  r2_b16a4x64f_vacccnt3_user_data_in/1 -> sim_out/1
  out_reg/1 -> assert_reg/1
  assert_reg/1 -> reint1/1
  reint1/1 -> io_delay/1

== system r2_b16a4x64f/vaccerr0 ==
  out_reg : Inport
  assert_reg : xbsIndex_r4/Assert  assert_type=on  type_source=Explicitly  gui_display_data_type=Fixed-point  arith_type=Unsigned  n_bits=16  bin_pt=0  preci_type=Single  exp_width=8  frac_width=24  assert_rate=off  rate_source=Explicitly  period=1  output_port=on  block_type=assert
  cast_gw : xbsIndex_r4/Convert  gui_display_data_type=Fixed-point  arith_type=Unsigned  n_bits=32  bin_pt=0  float_type=Single  exp_bits=8  fraction_bits=24  quantization=Truncate  overflow=Wrap  en=off  latency=0  dbl_ovrd=off  pipeline=off  block_type=convert
  io_delay : xbsIndex_r4/Delay  rst=off  infoeditControl=Selection of Reset will increase slice count due to use of real FFs and instead of SRLs  en=off  latency=1  dbl_ovrd=off  reg_retiming=on  block_type=delay
  r2_b16a4x64f_vaccerr0_user_data_in : xbsIndex_r4/Gateway Out  inherit_from_input=off  hdl_port=on  timing_constraint=None  locs_specified=off  LOCs={}  UseAsDAC=off  DACChannel='1'  block_type=gatewayout
  reint1 : xbsIndex_r4/Reinterpret  force_arith_type=on  arith_type=Unsigned  force_bin_pt=on  bin_pt=0  block_type=reinterpret
  sim_out : Terminator
  wires:
  io_delay/1 -> cast_gw/1
  cast_gw/1 -> r2_b16a4x64f_vaccerr0_user_data_in/1
  r2_b16a4x64f_vaccerr0_user_data_in/1 -> sim_out/1
  out_reg/1 -> assert_reg/1
  assert_reg/1 -> reint1/1
  reint1/1 -> io_delay/1

== system r2_b16a4x64f/vaccerr1 ==
  out_reg : Inport
  assert_reg : xbsIndex_r4/Assert  assert_type=on  type_source=Explicitly  gui_display_data_type=Fixed-point  arith_type=Unsigned  n_bits=16  bin_pt=0  preci_type=Single  exp_width=8  frac_width=24  assert_rate=off  rate_source=Explicitly  period=1  output_port=on  block_type=assert
  cast_gw : xbsIndex_r4/Convert  gui_display_data_type=Fixed-point  arith_type=Unsigned  n_bits=32  bin_pt=0  float_type=Single  exp_bits=8  fraction_bits=24  quantization=Truncate  overflow=Wrap  en=off  latency=0  dbl_ovrd=off  pipeline=off  block_type=convert
  io_delay : xbsIndex_r4/Delay  rst=off  infoeditControl=Selection of Reset will increase slice count due to use of real FFs and instead of SRLs  en=off  latency=1  dbl_ovrd=off  reg_retiming=on  block_type=delay
  r2_b16a4x64f_vaccerr1_user_data_in : xbsIndex_r4/Gateway Out  inherit_from_input=off  hdl_port=on  timing_constraint=None  locs_specified=off  LOCs={}  UseAsDAC=off  DACChannel='1'  block_type=gatewayout
  reint1 : xbsIndex_r4/Reinterpret  force_arith_type=on  arith_type=Unsigned  force_bin_pt=on  bin_pt=0  block_type=reinterpret
  sim_out : Terminator
  wires:
  io_delay/1 -> cast_gw/1
  cast_gw/1 -> r2_b16a4x64f_vaccerr1_user_data_in/1
  r2_b16a4x64f_vaccerr1_user_data_in/1 -> sim_out/1
  out_reg/1 -> assert_reg/1
  assert_reg/1 -> reint1/1
  reint1/1 -> io_delay/1

== system r2_b16a4x64f/vaccerr2 ==
  out_reg : Inport
  assert_reg : xbsIndex_r4/Assert  assert_type=on  type_source=Explicitly  gui_display_data_type=Fixed-point  arith_type=Unsigned  n_bits=16  bin_pt=0  preci_type=Single  exp_width=8  frac_width=24  assert_rate=off  rate_source=Explicitly  period=1  output_port=on  block_type=assert
  cast_gw : xbsIndex_r4/Convert  gui_display_data_type=Fixed-point  arith_type=Unsigned  n_bits=32  bin_pt=0  float_type=Single  exp_bits=8  fraction_bits=24  quantization=Truncate  overflow=Wrap  en=off  latency=0  dbl_ovrd=off  pipeline=off  block_type=convert
  io_delay : xbsIndex_r4/Delay  rst=off  infoeditControl=Selection of Reset will increase slice count due to use of real FFs and instead of SRLs  en=off  latency=1  dbl_ovrd=off  reg_retiming=on  block_type=delay
  r2_b16a4x64f_vaccerr2_user_data_in : xbsIndex_r4/Gateway Out  inherit_from_input=off  hdl_port=on  timing_constraint=None  locs_specified=off  LOCs={}  UseAsDAC=off  DACChannel='1'  block_type=gatewayout
  reint1 : xbsIndex_r4/Reinterpret  force_arith_type=on  arith_type=Unsigned  force_bin_pt=on  bin_pt=0  block_type=reinterpret
  sim_out : Terminator
  wires:
  io_delay/1 -> cast_gw/1
  cast_gw/1 -> r2_b16a4x64f_vaccerr2_user_data_in/1
  r2_b16a4x64f_vaccerr2_user_data_in/1 -> sim_out/1
  out_reg/1 -> assert_reg/1
  assert_reg/1 -> reint1/1
  reint1/1 -> io_delay/1

== system r2_b16a4x64f/vaccerr3 ==
  out_reg : Inport
  assert_reg : xbsIndex_r4/Assert  assert_type=on  type_source=Explicitly  gui_display_data_type=Fixed-point  arith_type=Unsigned  n_bits=16  bin_pt=0  preci_type=Single  exp_width=8  frac_width=24  assert_rate=off  rate_source=Explicitly  period=1  output_port=on  block_type=assert
  cast_gw : xbsIndex_r4/Convert  gui_display_data_type=Fixed-point  arith_type=Unsigned  n_bits=32  bin_pt=0  float_type=Single  exp_bits=8  fraction_bits=24  quantization=Truncate  overflow=Wrap  en=off  latency=0  dbl_ovrd=off  pipeline=off  block_type=convert
  io_delay : xbsIndex_r4/Delay  rst=off  infoeditControl=Selection of Reset will increase slice count due to use of real FFs and instead of SRLs  en=off  latency=1  dbl_ovrd=off  reg_retiming=on  block_type=delay
  r2_b16a4x64f_vaccerr3_user_data_in : xbsIndex_r4/Gateway Out  inherit_from_input=off  hdl_port=on  timing_constraint=None  locs_specified=off  LOCs={}  UseAsDAC=off  DACChannel='1'  block_type=gatewayout
  reint1 : xbsIndex_r4/Reinterpret  force_arith_type=on  arith_type=Unsigned  force_bin_pt=on  bin_pt=0  block_type=reinterpret
  sim_out : Terminator
  wires:
  io_delay/1 -> cast_gw/1
  cast_gw/1 -> r2_b16a4x64f_vaccerr3_user_data_in/1
  r2_b16a4x64f_vaccerr3_user_data_in/1 -> sim_out/1
  out_reg/1 -> assert_reg/1
  assert_reg/1 -> reint1/1
  reint1/1 -> io_delay/1
